simulink model "AEB_v1_wzq"  (R2025a)
settings: Solver=VariableStepAuto  StartTime=0.0  StopTime=10.0  RelTol=1e-3
libraries: simulink x1
settings Model: Creator=ziqi  LastModifiedBy=ziqi

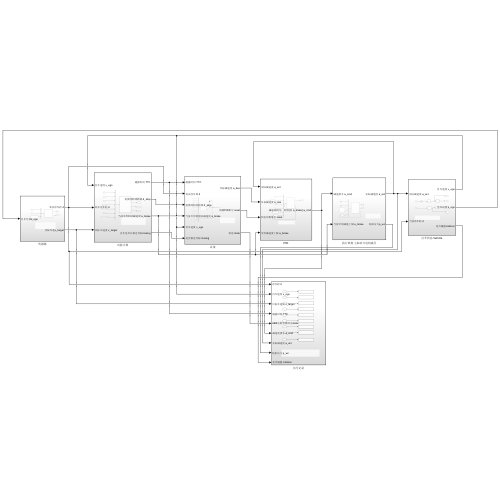
[thumbnail: Simulink's stored preview of the top-level diagram]
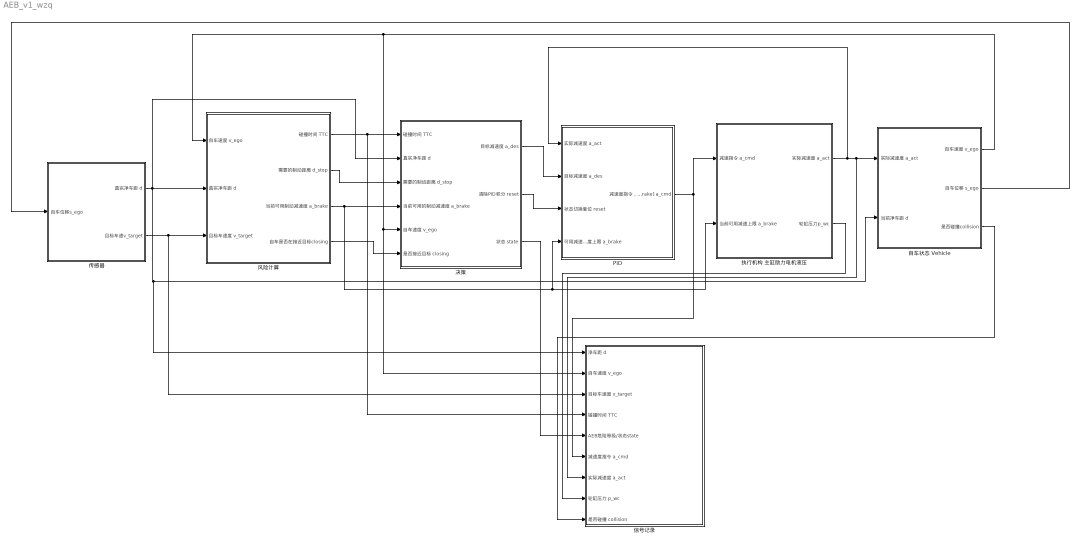
== system AEB_v1_wzq ==
  PID : Subsystem
  传感器 : Subsystem
  信号记录 : Subsystem
  决策 : Subsystem
  执行机构 主缸助力电机液压 : Subsystem
  自车状态 Vehicle : Subsystem
  风险计算 : Subsystem
  wires:
  自车状态 Vehicle/2(自车位移 s_ego) -> 传感器/1(自车位移s_ego)
  传感器/1(真实净车距 d) -> 信号记录/1(净车距 d), 自车状态 Vehicle/2(当前净车距 d), 决策/2(真实净车距 d), 风险计算/2(真实净车距 d)
  传感器/2(目标车速v_target) -> 信号记录/3(目标车速度 v_target), 风险计算/3(目标车速度 v_target)
  自车状态 Vehicle/1(自车速度 v_ego) -> 信号记录/2(自车速度 v_ego), 决策/5(自车速度 v_ego), 风险计算/1(自车速度 v_ego)
  风险计算/1(碰撞时间 TTC) -> 信号记录/4(碰撞时间 TTC), 决策/1(碰撞时间 TTC)
  风险计算/2(需要的制动距离 d_stop) -> 决策/3(需要的制动距离 d_stop)
  风险计算/3(当前可用制动减速度 a_brake) -> PID/4(可用减速度上限 a_brake), 执行机构 主缸助力电机液压/2(当前可用减速上限 a_brake), 决策/4(当前可用的制动减速度 a_brake)
  风险计算/4(自车是否在接近目标closing) -> 决策/6(是否接近目标 closing)
  决策/2(清除PID积分 reset) -> PID/3(状态切换复位 reset)
  决策/1(目标减速度 a_des) -> PID/2(目标减速度 a_des)
  PID/1("减速度指令，范围 [0, a_brake] a_cmd") -> 执行机构 主缸助力电机液压/1(减速指令 a_cmd), 信号记录/6(减速度指令 a_cmd)
  执行机构 主缸助力电机液压/1(实际减速度 a_act) -> 自车状态 Vehicle/1(实际减速度 a_act), 信号记录/7(实际减速度 a_act), PID/1(实际减速度 a_act)
  决策/3(状态 state) -> 信号记录/5(AEB危险等级/状态state)
  执行机构 主缸助力电机液压/2(轮缸压力p_wc) -> 信号记录/8(轮缸压力 p_wc)
  自车状态 Vehicle/3(是否碰撞collision) -> 信号记录/9(是否碰撞 collision)

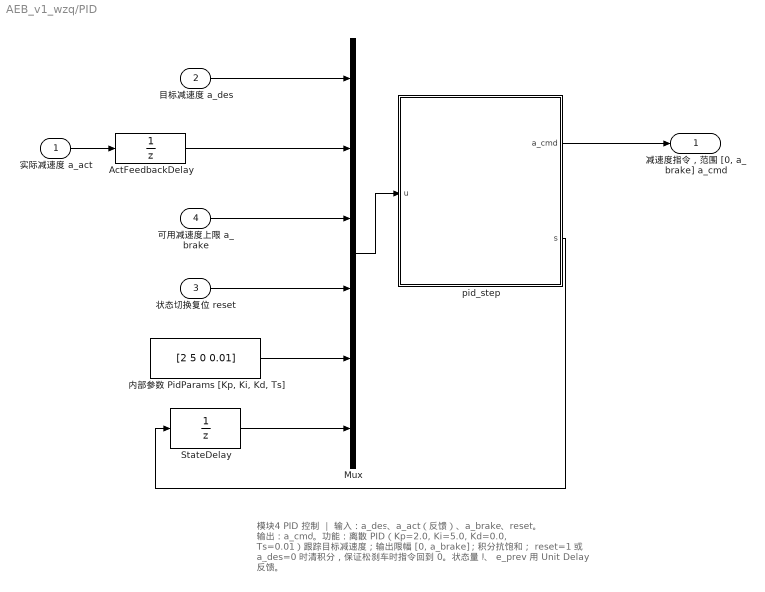
== system AEB_v1_wzq/PID ==
  note: 模块4 PID 控制 ｜ 输入：a_des、a_act（反馈）、a_brake、reset。
      | 输出：a_cmd。功能：离散 PID（Kp=2.0, Ki=5.0, Kd=0.0,
      | Ts=0.01）跟踪目标减速度；输出限幅 [0, a_brake]；积分抗饱和；
      | reset=1 或 a_des=0 时清积分，保证松刹车时指令回到 0。状态量 I、
      | e_prev 用 Unit Delay 反馈。
  实际减速度 a_act : Inport
  目标减速度 a_des : Inport  Port=2
  状态切换复位 reset : Inport  Port=3
  可用减速度上限 a_brake : Inport  Port=4
  ActFeedbackDelay : UnitDelay  SampleTime=0.01  HasFrameUpgradeWarning=on
  Mux : Mux  Inputs=6
  StateDelay : UnitDelay  InitialCondition=[0 0]  SampleTime=0.01  HasFrameUpgradeWarning=on
  pid_step : MATLAB Function  TreatAsAtomicUnit=on
  "内部参数 PidParams [Kp, Ki, Kd, Ts]" : Constant  Value=[2 5 0 0.01]
  "减速度指令，范围 [0, a_brake] a_cmd" : Outport
  wires:
  目标减速度 a_des/1 -> Mux/1
  实际减速度 a_act/1 -> ActFeedbackDelay/1
  ActFeedbackDelay/1 -> Mux/2
  可用减速度上限 a_brake/1 -> Mux/3
  状态切换复位 reset/1 -> Mux/4
  "内部参数 PidParams [Kp, Ki, Kd, Ts]"/1 -> Mux/5
  StateDelay/1 -> Mux/6
  Mux/1 -> pid_step/1(u)
  pid_step/1(a_cmd) -> "减速度指令，范围 [0, a_brake] a_cmd"/1
  pid_step/2(s) -> StateDelay/1

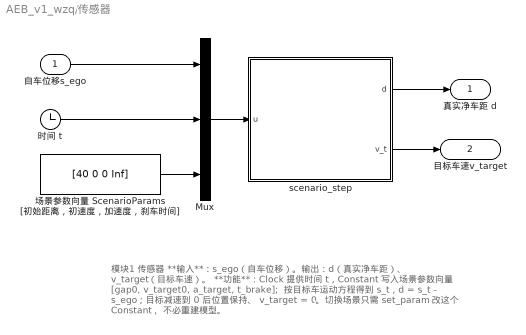
== system AEB_v1_wzq/传感器 ==
  note: 模块1 传感器
      | **输入**：s_ego（自车位移）。输出：d（真实净车距）、
      | v_target（目标车速）。
      | **功能**：Clock 提供时间 t，Constant
      | 写入场景参数向量 [gap0, v_target0, a_target, t_brake]；
      | 按目标车运动方程得到 s_t，d = s_t - s_ego；目标减速到 0 后位置保持、
      | v_target = 0。切换场景只需 set_param 改这个 Constant，
      | 不必重建模型。
  自车位移s_ego : Inport
  Mux : Mux  Inputs=3
  scenario_step : MATLAB Function  TreatAsAtomicUnit=on
  场景参数向量 ScenarioParams [初始距离，初速度，加速度，刹车时间] : Constant  Value=[40 0 0 Inf]
  时间 t : Clock
  真实净车距 d : Outport
  目标车速v_target : Outport  Port=2
  wires:
  自车位移s_ego/1 -> Mux/1
  时间 t/1 -> Mux/2
  场景参数向量 ScenarioParams [初始距离，初速度，加速度，刹车时间]/1 -> Mux/3
  Mux/1 -> scenario_step/1(u)
  scenario_step/1(d) -> 真实净车距 d/1
  scenario_step/2(v_t) -> 目标车速v_target/1

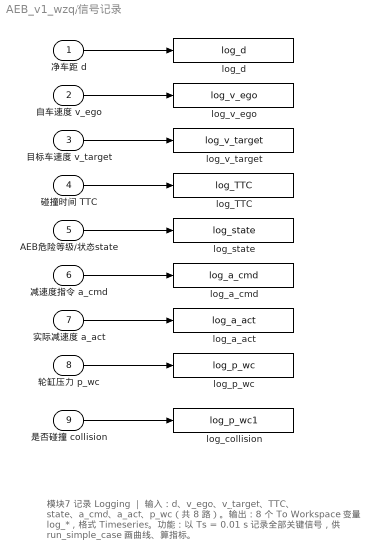
== system AEB_v1_wzq/信号记录 ==
  note: 模块7 记录 Logging ｜ 输入：d、v_ego、v_target、TTC、
      | state、a_cmd、a_act、p_wc（共 8 路）。输出：8 个 To
      | Workspace 变量 log_*，格式 Timeseries。功能：以 Ts =
      | 0.01 s 记录全部关键信号，供 run_simple_case 画曲线、算指标。
  净车距 d : Inport
  自车速度 v_ego : Inport  Port=2
  目标车速度 v_target : Inport  Port=3
  碰撞时间 TTC : Inport  Port=4
  AEB危险等级/状态state : Inport  Port=5
  减速度指令 a_cmd : Inport  Port=6
  实际减速度 a_act : Inport  Port=7
  轮缸压力 p_wc : Inport  Port=8
  是否碰撞 collision : Inport  Port=9
  log_TTC : ToWorkspace  VariableName=log_TTC  SaveFormat=Timeseries  SampleTime=0.01
  log_a_act : ToWorkspace  VariableName=log_a_act  SaveFormat=Timeseries  SampleTime=0.01
  log_a_cmd : ToWorkspace  VariableName=log_a_cmd  SaveFormat=Timeseries  SampleTime=0.01
  log_collision : ToWorkspace  VariableName=log_p_wc1  SaveFormat=Timeseries  SampleTime=0.01
  log_d : ToWorkspace  VariableName=log_d  SaveFormat=Timeseries  SampleTime=0.01
  log_p_wc : ToWorkspace  VariableName=log_p_wc  SaveFormat=Timeseries  SampleTime=0.01
  log_state : ToWorkspace  VariableName=log_state  SaveFormat=Timeseries  SampleTime=0.01
  log_v_ego : ToWorkspace  VariableName=log_v_ego  SaveFormat=Timeseries  SampleTime=0.01
  log_v_target : ToWorkspace  VariableName=log_v_target  SaveFormat=Timeseries  SampleTime=0.01
  wires:
  净车距 d/1 -> log_d/1
  自车速度 v_ego/1 -> log_v_ego/1
  目标车速度 v_target/1 -> log_v_target/1
  碰撞时间 TTC/1 -> log_TTC/1
  AEB危险等级/状态state/1 -> log_state/1
  减速度指令 a_cmd/1 -> log_a_cmd/1
  实际减速度 a_act/1 -> log_a_act/1
  轮缸压力 p_wc/1 -> log_p_wc/1
  是否碰撞 collision/1 -> log_collision/1

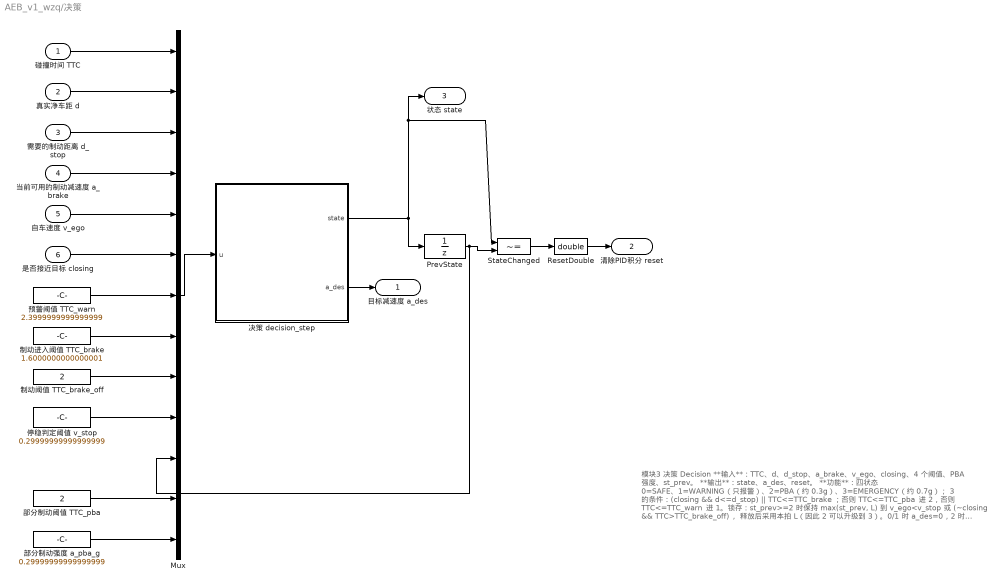
== system AEB_v1_wzq/决策 ==
  note: 模块3 决策 Decision
      | **输入**：TTC、d、d_stop、a_brake、v_ego、closing、4 个阈值、PBA 强度、st_prev。
      | **输出**：state、a_des、reset。
      | **功能**：四状态
      | 0=SAFE、1=WARNING（只报警）、2=PBA（约 0.3g）、3=EMERGENCY（约 0.7g）；
      | 3 的条件：(closing && d<=d_stop) || TTC<=TTC_brake；否则
      | TTC<=TTC_pba 进 2，否则 TTC<=TTC_warn 进 1。锁存：st_prev>=2 时保持
      | max(st_prev, L) 到 v_ego<v_stop 或 (~closing && TTC>TTC_brake_off)，
      | 释放后采用本拍 L（因此 2 可以升级到 3）。0/1 时 a_des=0，2 时
      | a_des=a_pba=min(a_pba_g*g, a_brake)，3 时 a_des=a_brake。
      | state 变化时 reset=1，供 PID 清积分。
  碰撞时间 TTC : Inport
  真实净车距 d : Inport  Port=2
  需要的制动距离 d_stop : Inport  Port=3
  当前可用的制动减速度 a_brake : Inport  Port=4
  自车速度 v_ego : Inport  Port=5
  是否接近目标 closing : Inport  Port=6
  " 停稳判定阈值 v_stop" : Constant  Value=0.29999999999999999
  Mux : Mux  Inputs=13
  PrevState : UnitDelay  SampleTime=0.01  HasFrameUpgradeWarning=on
  ResetDouble : DataTypeConversion  OutDataTypeStr=double  SaturateOnIntegerOverflow=off  RndMeth=Floor
  StateChanged : RelationalOperator  Operator=~=  OutDataTypeStr=boolean  RndMeth=Simplest  InputSameDT=off
  决策 decision_step : MATLAB Function  TreatAsAtomicUnit=on
  制动进入阈值 TTC_brake : Constant  Value=1.6000000000000001
  制动阈值 TTC_brake_off : Constant  Value=2
  部分制动强度 a_pba_g : Constant  Value=0.29999999999999999
  部分制动阈值 TTC_pba : Constant  Value=2
  预警阈值 TTC_warn : Constant  Value=2.3999999999999999
  目标减速度 a_des : Outport
  清除PID积分 reset : Outport  Port=2
  状态 state : Outport  Port=3
  wires:
  碰撞时间 TTC/1 -> Mux/1
  真实净车距 d/1 -> Mux/2
  需要的制动距离 d_stop/1 -> Mux/3
  当前可用的制动减速度 a_brake/1 -> Mux/4
  自车速度 v_ego/1 -> Mux/5
  是否接近目标 closing/1 -> Mux/6
  预警阈值 TTC_warn/1 -> Mux/7
  制动进入阈值 TTC_brake/1 -> Mux/8
  制动阈值 TTC_brake_off/1 -> Mux/9
  " 停稳判定阈值 v_stop"/1 -> Mux/10
  PrevState/1 -> Mux/11, StateChanged/2
  Mux/1 -> 决策 decision_step/1(u)
  决策 decision_step/1(state) -> 状态 state/1, StateChanged/1, PrevState/1
  决策 decision_step/2(a_des) -> 目标减速度 a_des/1
  StateChanged/1 -> ResetDouble/1
  ResetDouble/1 -> 清除PID积分 reset/1
  部分制动阈值 TTC_pba/1 -> Mux/12
  部分制动强度 a_pba_g/1 -> Mux/13

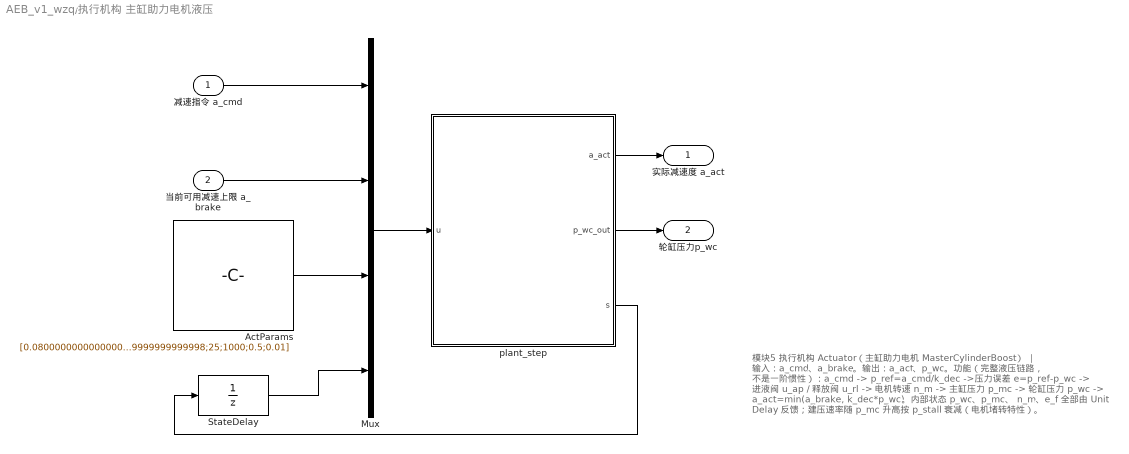
== system AEB_v1_wzq/执行机构 主缸助力电机液压 ==
  note: 模块5 执行机构 Actuator（主缸助力电机 MasterCylinderBoost）
      | ｜ 输入：a_cmd、a_brake。输出：a_act、p_wc。功能（完整液压链路，
      | 不是一阶惯性）：a_cmd -> p_ref=a_cmd/k_dec -> 压力误差
      | e=p_ref-p_wc -> 进液阀 u_ap / 释放阀 u_rl -> 电机转速
      | n_m -> 主缸压力 p_mc -> 轮缸压力 p_wc ->
      | a_act=min(a_brake, k_dec*p_wc)。内部状态 p_wc、p_mc、
      | n_m、e_f 全部由 Unit Delay 反馈；建压速率随 p_mc 升高按
      | p_stall 衰减（电机堵转特性）。
  减速指令 a_cmd : Inport
  当前可用减速上限 a_brake : Inport  Port=2
  ActParams : Constant  Value=[0.080000000000000002;1;180;0.040000000000000001;0.050000000000000003;0.01;0.02;0.29999999999999999;0.02;0.01;15;2500;0.059999999999999998;700;220;0.059999999999999998;25;1000;0.5;0.01]
  Mux : Mux
  StateDelay : UnitDelay  InitialCondition=[0;0;0;0]  SampleTime=0.01  HasFrameUpgradeWarning=on
  plant_step : MATLAB Function  TreatAsAtomicUnit=on
  实际减速度 a_act : Outport
  轮缸压力p_wc : Outport  Port=2
  wires:
  减速指令 a_cmd/1 -> Mux/1
  当前可用减速上限 a_brake/1 -> Mux/2
  ActParams/1 -> Mux/3
  StateDelay/1 -> Mux/4
  Mux/1 -> plant_step/1(u)
  plant_step/1(a_act) -> 实际减速度 a_act/1
  plant_step/2(p_wc_out) -> 轮缸压力p_wc/1
  plant_step/3(s) -> StateDelay/1

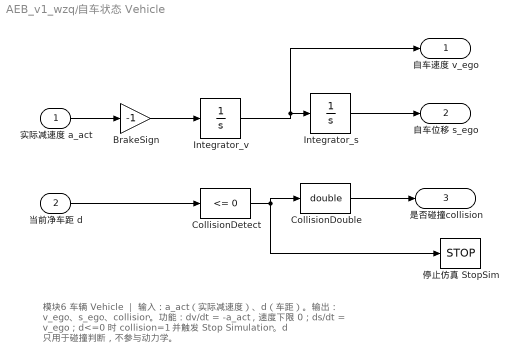
== system AEB_v1_wzq/自车状态 Vehicle ==
  note: 模块6 车辆 Vehicle ｜ 输入：a_act（实际减速度）、d（车距）。输出：
      | v_ego、s_ego、collision。功能：dv/dt = -a_act，速度下限
      | 0；ds/dt = v_ego；d<=0 时 collision=1 并触发 Stop
      | Simulation。d 只用于碰撞判断，不参与动力学。
  实际减速度 a_act : Inport
  当前净车距 d : Inport  Port=2
  BrakeSign : Gain  Gain=-1
  CollisionDetect : simulink/Logic and Bit Operations/Compare To Zero  relop=<=  OutDataTypeStr=boolean
  CollisionDouble : DataTypeConversion  OutDataTypeStr=double  SaturateOnIntegerOverflow=off  RndMeth=Floor
  Integrator_s : Integrator
  Integrator_v : Integrator  InitialCondition=11.111111111111111  LimitOutput=on  LowerSaturationLimit=0
  停止仿真 StopSim : Stop
  自车速度 v_ego : Outport
  自车位移 s_ego : Outport  Port=2
  是否碰撞collision : Outport  Port=3
  wires:
  实际减速度 a_act/1 -> BrakeSign/1
  BrakeSign/1 -> Integrator_v/1
  Integrator_v/1 -> Integrator_s/1, 自车速度 v_ego/1
  Integrator_s/1 -> 自车位移 s_ego/1
  当前净车距 d/1 -> CollisionDetect/1
  CollisionDetect/1 -> 停止仿真 StopSim/1, CollisionDouble/1
  CollisionDouble/1 -> 是否碰撞collision/1

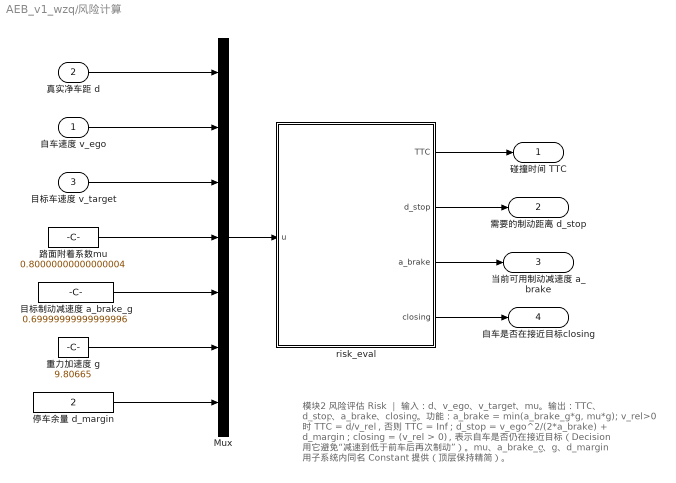
== system AEB_v1_wzq/风险计算 ==
  note: 模块2 风险评估 Risk ｜ 输入：d、v_ego、v_target、mu。输出：TTC、
      | d_stop、a_brake、closing。功能：a_brake =
      | min(a_brake_g*g, mu*g)；v_rel>0 时 TTC =
      | d/v_rel，否则 TTC = Inf；d_stop =
      | v_ego^2/(2*a_brake) + d_margin；closing =
      | (v_rel > 0)，表示自车是否仍在接近目标（Decision
      | 用它避免“减速到低于前车后再次制动”）。mu、a_brake_g、g、d_margin
      | 用子系统内同名 Constant 提供（顶层保持精简）。
  自车速度 v_ego : Inport
  真实净车距 d : Inport  Port=2
  目标车速度 v_target : Inport  Port=3
  Mux : Mux  Inputs=7
  risk_eval : MATLAB Function  TreatAsAtomicUnit=on
  停车余量 d_margin : Constant  Value=2
  目标制动减速度 a_brake_g : Constant  Value=0.69999999999999996
  路面附着系数mu : Constant  Value=0.80000000000000004
  重力加速度 g : Constant  Value=9.80665
  碰撞时间 TTC : Outport
  需要的制动距离 d_stop : Outport  Port=2
  当前可用制动减速度 a_brake : Outport  Port=3
  自车是否在接近目标closing : Outport  Port=4
  wires:
  真实净车距 d/1 -> Mux/1
  自车速度 v_ego/1 -> Mux/2
  目标车速度 v_target/1 -> Mux/3
  路面附着系数mu/1 -> Mux/4
  目标制动减速度 a_brake_g/1 -> Mux/5
  重力加速度 g/1 -> Mux/6
  停车余量 d_margin/1 -> Mux/7
  Mux/1 -> risk_eval/1(u)
  risk_eval/1(TTC) -> 碰撞时间 TTC/1
  risk_eval/2(d_stop) -> 需要的制动距离 d_stop/1
  risk_eval/3(a_brake) -> 当前可用制动减速度 a_brake/1
  risk_eval/4(closing) -> 自车是否在接近目标closing/1

== matlab function AEB_v1_wzq/风险计算/risk_eval ==
  settings: updateMethod=DISCRETE  sampleTime=0.01
  data: u input; TTC output; d_stop output; a_brake output; closing output
function [TTC, d_stop, a_brake, closing] = risk_eval(u)
% u = [d; v_ego; v_target; mu; a_brake_g; g; d_margin]
d = u(1);
ve = u(2);
vt = u(3);
mu = u(4);
abg = u(5);
g = u(6);
dm = u(7);
a_brake = min(abg * g, mu * g);
v_rel = ve - vt;
closing = double(v_rel > 0);
if v_rel > 0
    TTC = d / v_rel;
else
    TTC = Inf;
end
d_stop = ve * ve / (2 * a_brake) + dm;
end

== matlab function AEB_v1_wzq/传感器/scenario_step ==
  settings: updateMethod=DISCRETE  sampleTime=0.01
  data: u input; d output; v_t output
function [d, v_t] = scenario_step(u)
% Target vehicle motion and true gap (parameter driven).
% u = [s_ego; t; gap0; v_target0; a_target; t_brake]
s_ego = u(1);
t = u(2);
gap0 = u(3);
v0 = u(4);
at = u(5);
tb = u(6);
if t <= tb
    v_t = v0;
    s_t = gap0 + v0 * t;
else
    dt = t - tb;
    if at < 0 && (v0 + at * dt) <= 0
        t_stop = -v0 / at;
        s_t = gap0 + v0 * tb + v0 * t_stop ...
            + 0.5 * at * t_stop * t_stop;
        v_t = 0;
    else
        v_t = v0 + at * dt;
        s_t = gap0 + v0 * tb + v0 * dt + 0.5 * at * dt * dt;
    end
end
d = s_t - s_ego;
end

== matlab function AEB_v1_wzq/决策/决策 decision_step ==
  settings: updateMethod=DISCRETE  sampleTime=0.01
  data: u input; state output; a_des output
function [state, a_des] = decision_step(u)
% u = [TTC; d; d_stop; a_brake; v_ego; closing; TTC_warn;
%      TTC_brake; TTC_brake_off; v_stop; st_prev; TTC_pba; a_pba_g]
TTC = u(1);
d = u(2);
d_stop = u(3);
a_brake = u(4);
v_ego = u(5);
closing = u(6);
TTC_warn = u(7);
TTC_brake = u(8);
TTC_brake_off = u(9);
v_stop = u(10);
st_prev = u(11);
TTC_pba = u(12);
a_pba_g = u(13);
g = 9.80665;
a_pba = min(a_pba_g * g, a_brake);
% Four levels: 0 SAFE, 1 WARNING, 2 PBA, 3 EMERGENCY.
if (closing > 0.5 && d <= d_stop) || TTC <= TTC_brake
    L = 3;
elseif TTC <= TTC_pba
    L = 2;
elseif TTC <= TTC_warn
    L = 1;
else
    L = 0;
end
% Latch PBA/EMERGENCY: hold 2 or 3 until stopped, or until the target
% is no longer closing and TTC has recovered above TTC_brake_off.
st_prev = round(st_prev);
if st_prev >= 2
    if v_ego < v_stop || (closing < 0.5 && TTC > TTC_brake_off)
        state = L;
    else
        % Hold the higher of latched and current level, so PBA can
        % escalate to EMERGENCY without allowing 3 to drop early.
        state = max(st_prev, L);
    end
else
    state = L;
end
switch state
    case 3
        a_des = a_brake;
    case 2
        a_des = a_pba;
    otherwise
        a_des = 0;
end
end

== matlab function AEB_v1_wzq/PID/pid_step ==
  settings: updateMethod=DISCRETE  sampleTime=0.01
  data: u input; a_cmd output; s output
function [a_cmd, s] = pid_step(u)
% Discrete PID in velocity form with anti-windup.
% u = [a_des; a_act; a_brake; reset; Kp; Ki; Kd; Ts; I; e_prev]
a_des = u(1);
a_act = u(2);
a_brake = u(3);
reset = u(4);
Kp = u(5);
Ki = u(6);
Kd = u(7);
Ts = u(8);
I = u(9);
e_prev = u(10);
e = a_des - a_act;
if reset > 0.5 || a_des <= 0
    I = 0;
end
u_raw = Kp * e + Ki * I + Kd * (e - e_prev) / Ts;
u_sat = min(a_brake, max(0, u_raw));
% anti-windup: do not integrate when saturated further into the limit
if ~((u_raw > a_brake && e > 0) || (u_raw < 0 && e < 0))
    I_new = I + e * Ts;
else
    I_new = I;
end
a_cmd = u_sat;
s = [I_new, e];
end

== matlab function AEB_v1_wzq/执行机构 主缸助力电机液压/plant_step ==
  settings: updateMethod=DISCRETE  sampleTime=0.01
  data: u input; a_act output; p_wc_out output; s output
function [a_act, p_wc_out, s] = plant_step(u)
% Master-cylinder boost motor hydraulic plant (teaching model).
% u = [a_cmd; a_brake; p(1..20); p_wc; p_mc; n_m; e_f]
a_cmd = u(1);
a_brake = u(2);
p = u(3:22);
p_wc = u(23);
p_mc = u(24);
n_m = u(25);
e_f = u(26);
k_dec = p(1);
p_lp = p(2);
p_max = p(3);
tau_fill = p(4);
tau_rel = p(5);
Kv_ap = p(6);
Kv_rel = p(7);
e_db = p(8);
leak_wc = p(9);
Ts = p(10);
p_margin = p(11);
n_max = p(12);
tau_m = p(13);
p_build = p(14);
p_stall = p(15);
tau_use = p(16);
kp_n = p(17);
n_ff = p(18);
leak_mc = p(19);
tau_e = p(20);
% deceleration command -> wheel pressure target
p_ref = min(max(a_cmd, 0), a_brake) / k_dec;
% pressure error, filtered
e = p_ref - p_wc;
e_f_new = e_f + Ts * (e - e_f) / tau_e;
% apply / release valves
u_ap = 0;
u_rl = 0;
if e_f_new > e_db
    u_ap = min(1, max(0, Kv_ap * e_f_new));
elseif e_f_new < -e_db
    u_rl = min(1, max(0, Kv_rel * (-e_f_new)));
end
% boost motor speed loop: master-cylinder pressure follows p_ref + margin
n_cmd = min(n_max, max(0, kp_n * (p_ref + p_margin - p_mc) + n_ff));
n_new = n_m + Ts * (n_cmd - n_m) / tau_m;
n_new = min(n_max, max(-n_max, n_new));
% build rate falls as master-cylinder pressure approaches stall pressure
build_eff = p_build * max(0, 1 - p_mc / p_stall);
% master-cylinder pressure: motor build - flow to wheel - leak
dp_mc = (n_new / n_max) * build_eff ...
      - u_ap * max(p_mc - p_wc, 0) / tau_use ...
      - leak_mc * sign(max(p_mc - p_lp, 0));
% wheel-cylinder pressure: fill from master - release - leak
dp_wc = u_ap * max(p_mc - p_wc, 0) / tau_fill ...
      - u_rl * max(p_wc - p_lp, 0) / tau_rel ...
      - leak_wc * max(p_wc - p_lp, 0);
p_mc_new = min(p_max, max(0, p_mc + Ts * dp_mc));
p_wc_new = min(p_max, max(0, p_wc + Ts * dp_wc));
% a_act uses the *current state* p_wc, not p_wc_new, to avoid an
% algebraic loop with the PID in front of the plant.
a_act = min(a_brake, max(0, k_dec * p_wc));
p_wc_out = p_wc_new;
s = [p_wc_new; p_mc_new; n_new; e_f_new];
end
